simulink model "exp1"  (R2024a)
settings: Solver=VariableStepAuto  StartTime=0.0  StopTime=25  RelTol=1e-3
libraries: fl_lib x31, nesl_utility x16, ee_lib x6
settings Model: Creator=THEOFANIDIS  LastModifiedBy=Theof
settings DebuggingCC: UnconnectedInputMsg=warning  UnconnectedOutputMsg=warning  UnconnectedLineMsg=warning
settings ModelReferenceCC: EnableRefExpFcnMdlSchedulingChecks=on
settings RTWCC: GPUComputeCapability=3.5  DLArmComputeVersion=19.05

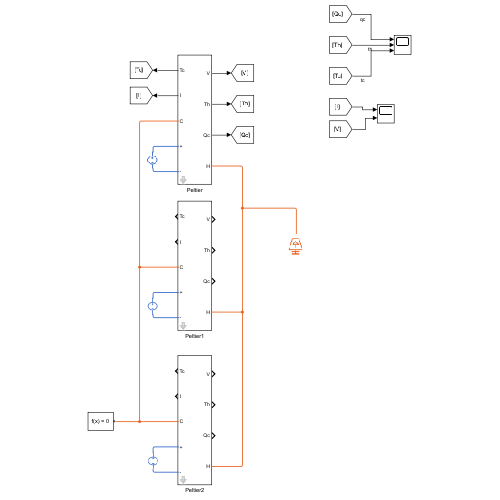
[thumbnail: Simulink's stored preview of the top-level diagram]
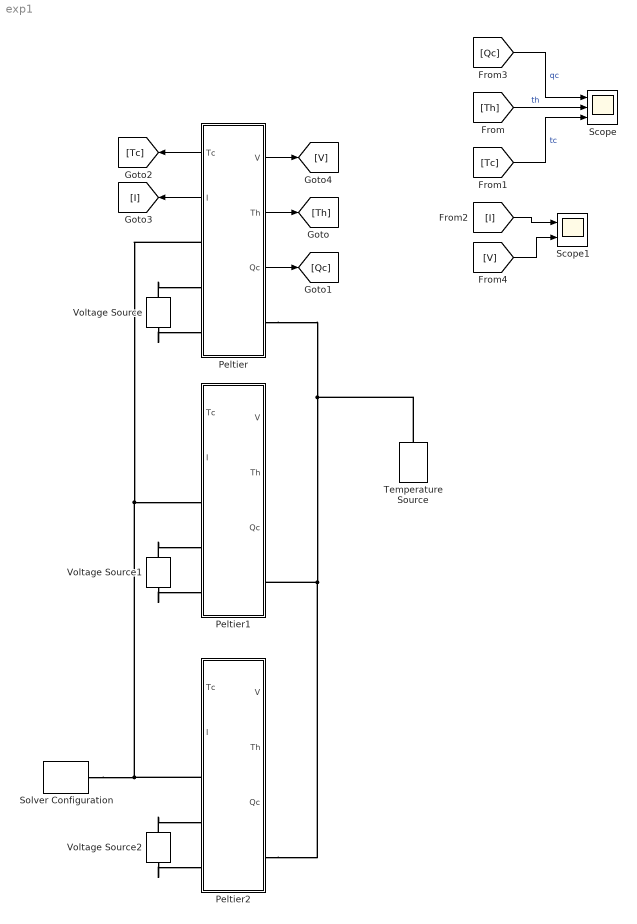
== system exp1 ==
  Peltier : Subsystem  mask{S=0.049, R=2.2, Rth=1.9, Cth=20}
      mask prompts: S "Seebeck coeff"; R "Resistance"; Rth "Thermal Resistance"; Cth "Thermal Capacity"
      settings: PortSchema="{\"entries\":[{\"content\":{\"sides\":[{\"content\":{\"connectorIds\":[\"Out4\",\"Out5\",\"LConn1\",\"LConn2\",\"LConn3\"]},\"type\":\"ConnectorPlacement.EquallySpacedRectSide\",\"uuid\":\"7b612d58-64a3-456b-8c94-0b47eb8aef96\"},{\"content\":{\"connectorIds\":[\"Out1\",\"Out2\",\"Out3\",\"RConn1\"],\"side\":\"RIGHT\"},\"type\":\"ConnectorPlacement.EquallySpacedRectSide\",\"uuid\":\"2f2d1fc6-4c28-432f-83e8-52c7cae39343\"},{\"content\":{\"connectorIds\":[],\"side\":\"TOP\"},\"type\":\"ConnectorPlacement.EquallySpacedRectSide\",\"uuid\":\"b65206c2-8afd-44bb-a455-6ebd5e3b3815\"}]},\"type\":\"ConnectorPlacement.EquallySpacedConnector\",\"uuid\":\"72c1d7be-9b5b-4c47-b998-86198d006e1c\"}],\"packageUris\":[\"http://schema.mathworks.com/mf0/Connector/R2020b\"],\"version\":\"1.0\"}"
  Peltier1 : Subsystem  mask{S=0.049, R=2.2, Rth=1.9, Cth=20}
      mask prompts: S "Seebeck coeff"; R "Resistance"; Rth "Thermal Resistance"; Cth "Thermal Capacity"
      settings: PortSchema="{\"entries\":[{\"content\":{\"sides\":[{\"content\":{\"connectorIds\":[\"Out4\",\"Out5\",\"LConn1\",\"LConn2\",\"LConn3\"]},\"type\":\"ConnectorPlacement.EquallySpacedRectSide\",\"uuid\":\"7b612d58-64a3-456b-8c94-0b47eb8aef96\"},{\"content\":{\"connectorIds\":[\"Out1\",\"Out2\",\"Out3\",\"RConn1\"],\"side\":\"RIGHT\"},\"type\":\"ConnectorPlacement.EquallySpacedRectSide\",\"uuid\":\"2f2d1fc6-4c28-432f-83e8-52c7cae39343\"},{\"content\":{\"connectorIds\":[],\"side\":\"TOP\"},\"type\":\"ConnectorPlacement.EquallySpacedRectSide\",\"uuid\":\"b65206c2-8afd-44bb-a455-6ebd5e3b3815\"}]},\"type\":\"ConnectorPlacement.EquallySpacedConnector\",\"uuid\":\"72c1d7be-9b5b-4c47-b998-86198d006e1c\"}],\"packageUris\":[\"http://schema.mathworks.com/mf0/Connector/R2020b\"],\"version\":\"1.0\"}"
  Peltier2 : Subsystem  mask{S=0.049, R=2.2, Rth=1.9, Cth=20}
      mask prompts: S "Seebeck coeff"; R "Resistance"; Rth "Thermal Resistance"; Cth "Thermal Capacity"
      settings: PortSchema="{\"entries\":[{\"content\":{\"sides\":[{\"content\":{\"connectorIds\":[\"Out4\",\"Out5\",\"LConn1\",\"LConn2\",\"LConn3\"]},\"type\":\"ConnectorPlacement.EquallySpacedRectSide\",\"uuid\":\"7b612d58-64a3-456b-8c94-0b47eb8aef96\"},{\"content\":{\"connectorIds\":[\"Out1\",\"Out2\",\"Out3\",\"RConn1\"],\"side\":\"RIGHT\"},\"type\":\"ConnectorPlacement.EquallySpacedRectSide\",\"uuid\":\"2f2d1fc6-4c28-432f-83e8-52c7cae39343\"},{\"content\":{\"connectorIds\":[],\"side\":\"TOP\"},\"type\":\"ConnectorPlacement.EquallySpacedRectSide\",\"uuid\":\"b65206c2-8afd-44bb-a455-6ebd5e3b3815\"}]},\"type\":\"ConnectorPlacement.EquallySpacedConnector\",\"uuid\":\"72c1d7be-9b5b-4c47-b998-86198d006e1c\"}],\"packageUris\":[\"http://schema.mathworks.com/mf0/Connector/R2020b\"],\"version\":\"1.0\"}"
  Scope : Scope  NumInputPorts=3
  Scope1 : Scope  NumInputPorts=2
  Solver Configuration : nesl_utility/Solver Configuration  PhysicalDomain=network_engine_domain  SubClassName=solver  LeftPortType=input  RightPortType=generic  Tones=[]  Harmonics=[]  SimulateNoise=off  Profile=off  UseLocalSampling=off  EnableSwitchedLinearOptims=on  FrequencyDomain=off  UseCCode=off  RelTol=0.001  AbsTol=1e-06  MinStep=1e-09  ToWorkspace=off  RevertToSquareIcSolve=off  NumHomotopyIterations=100  PhasorMode=off  PhasorModeNumHarmonics=1  ConsistencySolver=NEWTON_FTOL  IndexReductionMethod=DerivativeReplacement  DoDC=off  ResidualTolerance=1e-09  ConsistencyTolSource=GLOBAL  ConsistencyAbsTol=0.001  ConsistencyRelTol=0.001  ConsistencyTolFactor=0.001  UseLocalSolver=off  LocalSolverChoice=NE_BACKWARD_EULER_ADVANCER  ResolveIndetEquations=on  FunctionEvalNumThread=1  LocalSolverSampleTime=0.001  DoFixedCost=off  MaxNonlinIter=3  MaxModeIter=2  ComputeImpulses=off  ImpulseIterations=2  LinearAlgebra=auto  LinearAlgebraNumThread=0  EquationFormulation=NE_TIME_EF  DelaysMemoryBudget=1024  AutomaticFiltering=on  FilteringTimeConstant=0.001  PartitionStorageMethod=AS_NEEDED  PartitionMemoryBudget=1024  PartitionMethod=ROBUST  MultibodyUseLocalSolver=off  MultibodyLocalSolverChoice=ODE1  MultibodyLocalSolverSampleTime=0.001
  Temperature Source : fl_lib/Thermal/Thermal Sources/Temperature Source  temperature=50 degC
  Voltage Source : ee_lib/Sources/Voltage Source  dc_voltage=12 V  ac_voltage=0 V  ac_shift=0 rad  ac_frequency=60 Hz  noise_mode=0  PSD=0 V^2/Hz  sample_time=1e-3 s  repeatability=1  user_seed=0  auto_seed=785646024  i_specify=off  i_priority=None  i=0 A  i_nominal_specify=off  i_nominal_value=1  i_nominal_unit=A  v_specify=off  v_priority=None  v=0 V  v_nominal_specify=off  v_nominal_value=1  v_nominal_unit=V
  Voltage Source1 : ee_lib/Sources/Voltage Source  dc_voltage=12 V  ac_voltage=0 V  ac_shift=0 rad  ac_frequency=60 Hz  noise_mode=0  PSD=0 V^2/Hz  sample_time=1e-3 s  repeatability=1  user_seed=0  auto_seed=3499211588  i_specify=off  i_priority=None  i=0 A  i_nominal_specify=off  i_nominal_value=1  i_nominal_unit=A  v_specify=off  v_priority=None  v=0 V  v_nominal_specify=off  v_nominal_value=1  v_nominal_unit=V
  Voltage Source2 : ee_lib/Sources/Voltage Source  dc_voltage=12 V  ac_voltage=0 V  ac_shift=0 rad  ac_frequency=60 Hz  noise_mode=0  PSD=0 V^2/Hz  sample_time=1e-3 s  repeatability=1  user_seed=0  auto_seed=3890346746  i_specify=off  i_priority=None  i=0 A  i_nominal_specify=off  i_nominal_value=1  i_nominal_unit=A  v_specify=off  v_priority=None  v=0 V  v_nominal_specify=off  v_nominal_value=1  v_nominal_unit=V
  wires:
  Peltier/2(Th) -> [Th]
  Peltier/3(Qc) -> [Qc]
  Peltier/4(Tc) -> [Tc]
  Peltier/5(I) -> [I]
  [Th] -> Scope/2  "th"
  [Tc] -> Scope/3  "tc"
  [Qc] -> Scope/1  "qc"
  Peltier/1(V) -> [V]
  [I] -> Scope1/1
  [V] -> Scope1/2
  connections:
  Voltage Source/LConn1 -- Peltier/LConn2
  Voltage Source/RConn1 -- Peltier/LConn3
  Voltage Source1/LConn1 -- Peltier1/LConn2
  Voltage Source1/RConn1 -- Peltier1/LConn3
  Voltage Source2/LConn1 -- Peltier2/LConn2
  Voltage Source2/RConn1 -- Peltier2/LConn3
  Peltier/RConn1 -- Temperature Source/LConn1 -- Peltier2/RConn1 -- Peltier1/RConn1
  Peltier2/LConn1 -- Solver Configuration/RConn1 -- Peltier/LConn1 -- Peltier1/LConn1

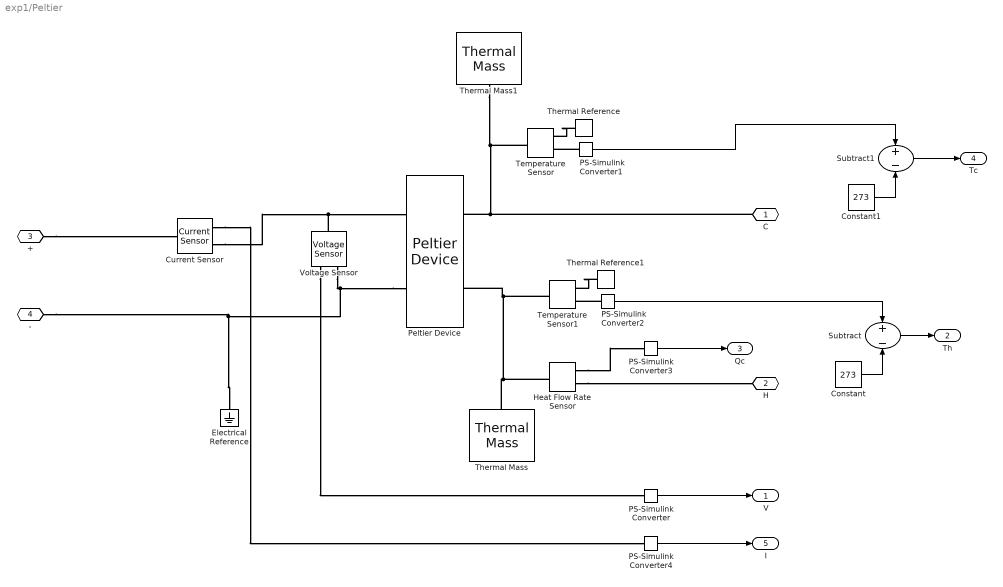
== system exp1/Peltier ==
  Constant : Constant  Value=273
  Constant1 : Constant  Value=273
  Current Sensor : fl_lib/Electrical/Electrical Sensors/Current Sensor
  Electrical Reference : fl_lib/Electrical/Electrical Elements/Electrical Reference
  Heat Flow Rate Sensor : fl_lib/Thermal/Thermal Sensors/Heat Flow Rate Sensor
  PS-Simulink Converter{,1..4} (5 alike) : nesl_utility/PS-Simulink Converter  PhysicalDomain=network_engine_domain  SubClassName=ps_output  LeftPortType=input  RightPortType=output  PseudoPeriodic=off  Frequencies=[]  VectorFormat=1-D array  Unit=inherit  AffineConversion=off
  Peltier Device : ee_lib/Sensors & Transducers/Peltier Device  alpha=S V/K  R=R Ohm  K=1/Rth W/K
      settings: InternalSimscapePortConfiguration="{\"Bottom\":[],\"Left\":[{\"id\":\"p\",\"label\":\"+\",\"type\":\"foundation.electrical.electrical\"},{\"id\":\"n\",\"label\":\"-\",\"type\":\"foundation.electrical.electrical\"}],\"Right\":[{\"id\":\"A\",\"label\":\"A\",\"type\":\"foundation.thermal.thermal\"},{\"id\":\"B\",\"label\":\"B\",\"type\":\"foundation.thermal.thermal\"}],\"Top\":[]}"
  Subtract : Sum  Inputs=+-
  Subtract1 : Sum  Inputs=+-
  Temperature Sensor : fl_lib/Thermal/Thermal Sensors/Temperature Sensor  temperature_measure=foundation.enum.MeasurementReference.difference
  Temperature Sensor1 : fl_lib/Thermal/Thermal Sensors/Temperature Sensor  temperature_measure=foundation.enum.MeasurementReference.difference
  Thermal Mass : fl_lib/Thermal/Thermal Elements/Thermal Mass  mass_type=foundation.enum.constant_variable.constant  mass=12 g  sp_heat=Cth/2/0.012 J/(K*kg)  mass_min=1e-6 kg  num_ports=foundation.enum.numPorts2.one  m_specify=off  m_priority=High  m=1 kg  m_nominal_specify=off  m_nominal_value=1  m_nominal_unit=kg  T_specify=off  T_priority=High  T=300 K  T_nominal_specify=off  T_nominal_value=1  T_nominal_unit=K  Q_specify=off  Q_priority=None  Q=0 W  Q_nominal_specify=off  Q_nominal_value=1  Q_nominal_unit=W
  Thermal Mass1 : fl_lib/Thermal/Thermal Elements/Thermal Mass  mass_type=foundation.enum.constant_variable.constant  mass=12 g  sp_heat=Cth/2/0.012 J/(K*kg)  mass_min=1e-6 kg  num_ports=foundation.enum.numPorts2.one  m_specify=off  m_priority=High  m=1 kg  m_nominal_specify=off  m_nominal_value=1  m_nominal_unit=kg  T_specify=off  T_priority=High  T=300 K  T_nominal_specify=off  T_nominal_value=1  T_nominal_unit=K  Q_specify=off  Q_priority=None  Q=0 W  Q_nominal_specify=off  Q_nominal_value=1  Q_nominal_unit=W
  Thermal Reference : fl_lib/Thermal/Thermal Elements/Thermal Reference
  Thermal Reference1 : fl_lib/Thermal/Thermal Elements/Thermal Reference
  Voltage Sensor : fl_lib/Electrical/Electrical Sensors/Voltage Sensor
  C : PMIOPort  Side=Left
  H : PMIOPort  Port=2  Side=Right
  + : PMIOPort  Port=3  Side=Left
  - : PMIOPort  Port=4  Side=Left
  V : Outport
  Th : Outport  Port=2
  Qc : Outport  Port=3
  Tc : Outport  Port=4
  I : Outport  Port=5
  wires:
  PS-Simulink Converter/1 -> V/1
  PS-Simulink Converter4/1 -> I/1
  Constant/1 -> Subtract/2
  PS-Simulink Converter2/1 -> Subtract/1
  Subtract/1 -> Th/1
  PS-Simulink Converter3/1 -> Qc/1
  Subtract1/1 -> Tc/1
  PS-Simulink Converter1/1 -> Subtract1/1
  Constant1/1 -> Subtract1/2
  connections:
  Voltage Sensor/RConn1 -- PS-Simulink Converter/LConn1
  Current Sensor/RConn2 -- Voltage Sensor/LConn1 -- Peltier Device/LConn1
  C/RConn1 -- Peltier Device/RConn1 -- Temperature Sensor/LConn1 -- Thermal Mass1/LConn1
  Heat Flow Rate Sensor/RConn1 -- PS-Simulink Converter3/LConn1
  Temperature Sensor1/LConn1 -- Peltier Device/RConn2 -- Heat Flow Rate Sensor/LConn1 -- Thermal Mass/LConn1
  Thermal Reference/LConn1 -- Temperature Sensor/RConn1
  PS-Simulink Converter1/LConn1 -- Temperature Sensor/RConn2
  PS-Simulink Converter2/LConn1 -- Temperature Sensor1/RConn2
  Thermal Reference1/LConn1 -- Temperature Sensor1/RConn1
  Heat Flow Rate Sensor/RConn2 -- H/RConn1
  Peltier Device/LConn2 -- Voltage Sensor/RConn2 -- Electrical Reference/LConn1 -- -/RConn1
  +/RConn1 -- Current Sensor/LConn1
  Current Sensor/RConn1 -- PS-Simulink Converter4/LConn1

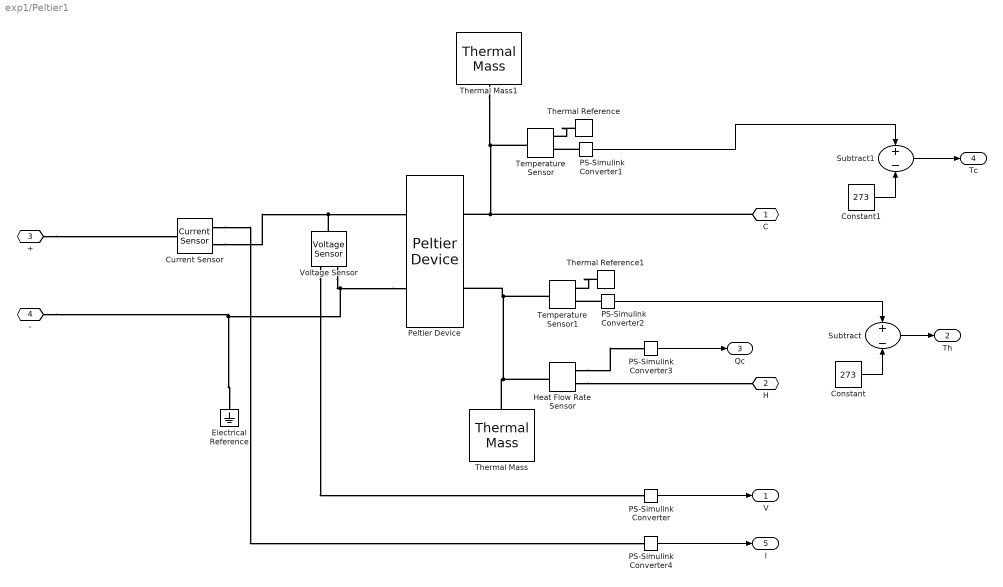
== system exp1/Peltier1 ==
  Constant : Constant  Value=273
  Constant1 : Constant  Value=273
  Current Sensor : fl_lib/Electrical/Electrical Sensors/Current Sensor
  Electrical Reference : fl_lib/Electrical/Electrical Elements/Electrical Reference
  Heat Flow Rate Sensor : fl_lib/Thermal/Thermal Sensors/Heat Flow Rate Sensor
  PS-Simulink Converter{,1..4} (5 alike) : nesl_utility/PS-Simulink Converter  PhysicalDomain=network_engine_domain  SubClassName=ps_output  LeftPortType=input  RightPortType=output  PseudoPeriodic=off  Frequencies=[]  VectorFormat=1-D array  Unit=inherit  AffineConversion=off
  Peltier Device : ee_lib/Sensors & Transducers/Peltier Device  alpha=S V/K  R=R Ohm  K=1/Rth W/K
      settings: InternalSimscapePortConfiguration="{\"Bottom\":[],\"Left\":[{\"id\":\"p\",\"label\":\"+\",\"type\":\"foundation.electrical.electrical\"},{\"id\":\"n\",\"label\":\"-\",\"type\":\"foundation.electrical.electrical\"}],\"Right\":[{\"id\":\"A\",\"label\":\"A\",\"type\":\"foundation.thermal.thermal\"},{\"id\":\"B\",\"label\":\"B\",\"type\":\"foundation.thermal.thermal\"}],\"Top\":[]}"
  Subtract : Sum  Inputs=+-
  Subtract1 : Sum  Inputs=+-
  Temperature Sensor : fl_lib/Thermal/Thermal Sensors/Temperature Sensor  temperature_measure=foundation.enum.MeasurementReference.difference
  Temperature Sensor1 : fl_lib/Thermal/Thermal Sensors/Temperature Sensor  temperature_measure=foundation.enum.MeasurementReference.difference
  Thermal Mass : fl_lib/Thermal/Thermal Elements/Thermal Mass  mass_type=foundation.enum.constant_variable.constant  mass=12 g  sp_heat=Cth/2/0.012 J/(K*kg)  mass_min=1e-6 kg  num_ports=foundation.enum.numPorts2.one  m_specify=off  m_priority=High  m=1 kg  m_nominal_specify=off  m_nominal_value=1  m_nominal_unit=kg  T_specify=off  T_priority=High  T=300 K  T_nominal_specify=off  T_nominal_value=1  T_nominal_unit=K  Q_specify=off  Q_priority=None  Q=0 W  Q_nominal_specify=off  Q_nominal_value=1  Q_nominal_unit=W
  Thermal Mass1 : fl_lib/Thermal/Thermal Elements/Thermal Mass  mass_type=foundation.enum.constant_variable.constant  mass=12 g  sp_heat=Cth/2/0.012 J/(K*kg)  mass_min=1e-6 kg  num_ports=foundation.enum.numPorts2.one  m_specify=off  m_priority=High  m=1 kg  m_nominal_specify=off  m_nominal_value=1  m_nominal_unit=kg  T_specify=off  T_priority=High  T=300 K  T_nominal_specify=off  T_nominal_value=1  T_nominal_unit=K  Q_specify=off  Q_priority=None  Q=0 W  Q_nominal_specify=off  Q_nominal_value=1  Q_nominal_unit=W
  Thermal Reference : fl_lib/Thermal/Thermal Elements/Thermal Reference
  Thermal Reference1 : fl_lib/Thermal/Thermal Elements/Thermal Reference
  Voltage Sensor : fl_lib/Electrical/Electrical Sensors/Voltage Sensor
  C : PMIOPort  Side=Left
  H : PMIOPort  Port=2  Side=Right
  + : PMIOPort  Port=3  Side=Left
  - : PMIOPort  Port=4  Side=Left
  V : Outport
  Th : Outport  Port=2
  Qc : Outport  Port=3
  Tc : Outport  Port=4
  I : Outport  Port=5
  wires:
  PS-Simulink Converter/1 -> V/1
  PS-Simulink Converter4/1 -> I/1
  Constant/1 -> Subtract/2
  PS-Simulink Converter2/1 -> Subtract/1
  Subtract/1 -> Th/1
  PS-Simulink Converter3/1 -> Qc/1
  Subtract1/1 -> Tc/1
  PS-Simulink Converter1/1 -> Subtract1/1
  Constant1/1 -> Subtract1/2
  connections:
  Voltage Sensor/RConn1 -- PS-Simulink Converter/LConn1
  Current Sensor/RConn2 -- Voltage Sensor/LConn1 -- Peltier Device/LConn1
  C/RConn1 -- Peltier Device/RConn1 -- Temperature Sensor/LConn1 -- Thermal Mass1/LConn1
  Heat Flow Rate Sensor/RConn1 -- PS-Simulink Converter3/LConn1
  Temperature Sensor1/LConn1 -- Peltier Device/RConn2 -- Heat Flow Rate Sensor/LConn1 -- Thermal Mass/LConn1
  Thermal Reference/LConn1 -- Temperature Sensor/RConn1
  PS-Simulink Converter1/LConn1 -- Temperature Sensor/RConn2
  PS-Simulink Converter2/LConn1 -- Temperature Sensor1/RConn2
  Thermal Reference1/LConn1 -- Temperature Sensor1/RConn1
  Heat Flow Rate Sensor/RConn2 -- H/RConn1
  Peltier Device/LConn2 -- Voltage Sensor/RConn2 -- Electrical Reference/LConn1 -- -/RConn1
  +/RConn1 -- Current Sensor/LConn1
  Current Sensor/RConn1 -- PS-Simulink Converter4/LConn1

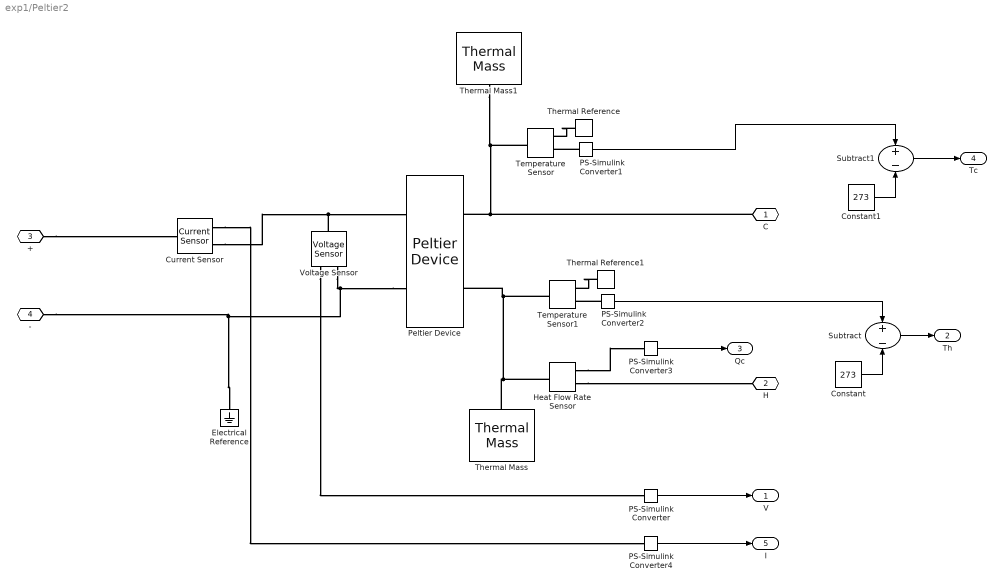
== system exp1/Peltier2 ==
  Constant : Constant  Value=273
  Constant1 : Constant  Value=273
  Current Sensor : fl_lib/Electrical/Electrical Sensors/Current Sensor
  Electrical Reference : fl_lib/Electrical/Electrical Elements/Electrical Reference
  Heat Flow Rate Sensor : fl_lib/Thermal/Thermal Sensors/Heat Flow Rate Sensor
  PS-Simulink Converter{,1..4} (5 alike) : nesl_utility/PS-Simulink Converter  PhysicalDomain=network_engine_domain  SubClassName=ps_output  LeftPortType=input  RightPortType=output  PseudoPeriodic=off  Frequencies=[]  VectorFormat=1-D array  Unit=inherit  AffineConversion=off
  Peltier Device : ee_lib/Sensors & Transducers/Peltier Device  alpha=S V/K  R=R Ohm  K=1/Rth W/K
      settings: InternalSimscapePortConfiguration="{\"Bottom\":[],\"Left\":[{\"id\":\"p\",\"label\":\"+\",\"type\":\"foundation.electrical.electrical\"},{\"id\":\"n\",\"label\":\"-\",\"type\":\"foundation.electrical.electrical\"}],\"Right\":[{\"id\":\"A\",\"label\":\"A\",\"type\":\"foundation.thermal.thermal\"},{\"id\":\"B\",\"label\":\"B\",\"type\":\"foundation.thermal.thermal\"}],\"Top\":[]}"
  Subtract : Sum  Inputs=+-
  Subtract1 : Sum  Inputs=+-
  Temperature Sensor : fl_lib/Thermal/Thermal Sensors/Temperature Sensor  temperature_measure=foundation.enum.MeasurementReference.difference
  Temperature Sensor1 : fl_lib/Thermal/Thermal Sensors/Temperature Sensor  temperature_measure=foundation.enum.MeasurementReference.difference
  Thermal Mass : fl_lib/Thermal/Thermal Elements/Thermal Mass  mass_type=foundation.enum.constant_variable.constant  mass=12 g  sp_heat=Cth/2/0.012 J/(K*kg)  mass_min=1e-6 kg  num_ports=foundation.enum.numPorts2.one  m_specify=off  m_priority=High  m=1 kg  m_nominal_specify=off  m_nominal_value=1  m_nominal_unit=kg  T_specify=off  T_priority=High  T=300 K  T_nominal_specify=off  T_nominal_value=1  T_nominal_unit=K  Q_specify=off  Q_priority=None  Q=0 W  Q_nominal_specify=off  Q_nominal_value=1  Q_nominal_unit=W
  Thermal Mass1 : fl_lib/Thermal/Thermal Elements/Thermal Mass  mass_type=foundation.enum.constant_variable.constant  mass=12 g  sp_heat=Cth/2/0.012 J/(K*kg)  mass_min=1e-6 kg  num_ports=foundation.enum.numPorts2.one  m_specify=off  m_priority=High  m=1 kg  m_nominal_specify=off  m_nominal_value=1  m_nominal_unit=kg  T_specify=off  T_priority=High  T=300 K  T_nominal_specify=off  T_nominal_value=1  T_nominal_unit=K  Q_specify=off  Q_priority=None  Q=0 W  Q_nominal_specify=off  Q_nominal_value=1  Q_nominal_unit=W
  Thermal Reference : fl_lib/Thermal/Thermal Elements/Thermal Reference
  Thermal Reference1 : fl_lib/Thermal/Thermal Elements/Thermal Reference
  Voltage Sensor : fl_lib/Electrical/Electrical Sensors/Voltage Sensor
  C : PMIOPort  Side=Left
  H : PMIOPort  Port=2  Side=Right
  + : PMIOPort  Port=3  Side=Left
  - : PMIOPort  Port=4  Side=Left
  V : Outport
  Th : Outport  Port=2
  Qc : Outport  Port=3
  Tc : Outport  Port=4
  I : Outport  Port=5
  wires:
  PS-Simulink Converter/1 -> V/1
  PS-Simulink Converter4/1 -> I/1
  Constant/1 -> Subtract/2
  PS-Simulink Converter2/1 -> Subtract/1
  Subtract/1 -> Th/1
  PS-Simulink Converter3/1 -> Qc/1
  Subtract1/1 -> Tc/1
  PS-Simulink Converter1/1 -> Subtract1/1
  Constant1/1 -> Subtract1/2
  connections:
  Voltage Sensor/RConn1 -- PS-Simulink Converter/LConn1
  Current Sensor/RConn2 -- Voltage Sensor/LConn1 -- Peltier Device/LConn1
  C/RConn1 -- Peltier Device/RConn1 -- Temperature Sensor/LConn1 -- Thermal Mass1/LConn1
  Heat Flow Rate Sensor/RConn1 -- PS-Simulink Converter3/LConn1
  Temperature Sensor1/LConn1 -- Peltier Device/RConn2 -- Heat Flow Rate Sensor/LConn1 -- Thermal Mass/LConn1
  Thermal Reference/LConn1 -- Temperature Sensor/RConn1
  PS-Simulink Converter1/LConn1 -- Temperature Sensor/RConn2
  PS-Simulink Converter2/LConn1 -- Temperature Sensor1/RConn2
  Thermal Reference1/LConn1 -- Temperature Sensor1/RConn1
  Heat Flow Rate Sensor/RConn2 -- H/RConn1
  Peltier Device/LConn2 -- Voltage Sensor/RConn2 -- Electrical Reference/LConn1 -- -/RConn1
  +/RConn1 -- Current Sensor/LConn1
  Current Sensor/RConn1 -- PS-Simulink Converter4/LConn1
